simulink model "RL_voltageControl"  (R2026a)
settings: Solver=VariableStepAuto  StopTime=2000  FixedStep=1e-5
libraries: fl_lib x3, nesl_utility x3, ee_lib x2, eePwmGenerator x1
settings Model: Creator=abhinav  LastModifiedBy=abhinav
settings DataIOCC: SaveFormat=StructureWithTime

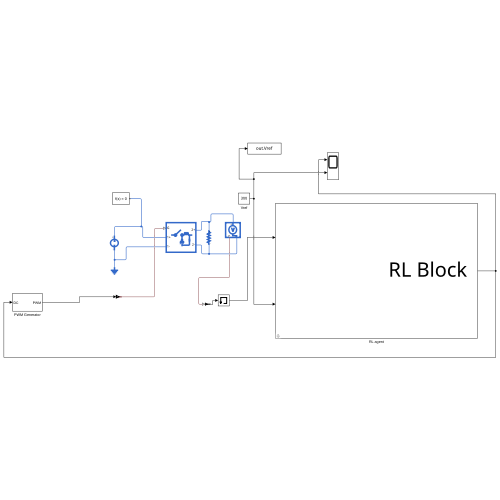
[thumbnail: Simulink's stored preview of the top-level diagram]
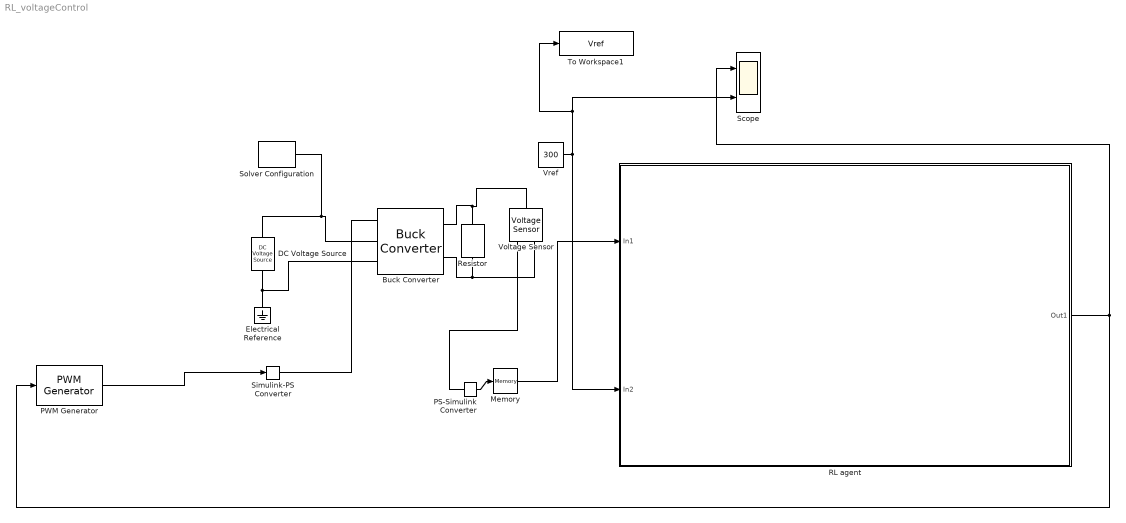
== system RL_voltageControl ==
  Buck Converter : ee_lib/Semiconductors & Converters/Converters/Buck Converter  port_option=ee.enum.controlport.ps  device_type=ee.enum.converters.switchingdevice.ideal  Vf=0.8 V  Ron=0.001 Ohm  Rds=0.001 Ohm  Goff=1e-5 1/Ohm  Vgt=1 V  Vgt_off=-1 V  Ih=1 A  Vth=6 V  K=0  diode_param=ee.enum.converters.protectiondiode.nodynamics  diode_Vf=0.8 V  diode_Ron=0.001 Ohm  diode_Goff=1e-5 1/Ohm  diode_C=50 nF  diode_iRM=-235 A  diode_iF=300 A  diode_idot=-50 A/us  diode_trr_param=ee.enum.converters.diodetrr.trr_factor  diode_trr_factor=3  diode_trr=15 us  diode_Qrr=1500 s*uA  Lf=1e-6 H  Rl=0 Ohm  Cf=1e-7 F  Rf=1e-6 Ohm  snubber_type=ee.enum.converters.snubber.exclude  Cs=1e-7 F  Rs=0.1 Ohm  iL_specify=off  iL_priority=High  iL=0 A  iL_nominal_specify=off  iL_nominal_value=1  iL_nominal_unit=A  vc_specify=off  vc_priority=High  vc=0 V  vc_nominal_specify=off  vc_nominal_value=1  vc_nominal_unit=V
  DC Voltage Source : ee_lib/Additional Components/SPICE Sources/DC Voltage Source  DC=500 V
  Electrical Reference : fl_lib/Electrical/Electrical Elements/Electrical Reference
  Memory : Memory
  PS-Simulink Converter : nesl_utility/PS-Simulink Converter  PhysicalDomain=network_engine_domain  SubClassName=ps_output  LeftPortType=input  RightPortType=output  PseudoPeriodic=off  Frequencies=[]  VectorFormat=inherit  Unit=inherit  AffineConversion=off
  PWM Generator : eePwmGenerator/PWM Generator  CarrCount=Up  Tper=0.01  Tdelay=0  Ts=1e-5
  RL agent : Subsystem  mask{Parameter1=0}
  Resistor : fl_lib/Electrical/Electrical Elements/Resistor  R=1 Ohm  i_specify=off  i_priority=None  i=0 A  i_nominal_specify=off  i_nominal_value=1  i_nominal_unit=A  v_specify=off  v_priority=None  v=0 V  v_nominal_specify=off  v_nominal_value=1  v_nominal_unit=V
  Scope : Scope  NumInputPorts=2
      settings: ActiveDisplayYMinimum=154.82767756144224  ActiveDisplayYMaximum=316.13025804872865
  Simulink-PS Converter : nesl_utility/Simulink-PS Converter  PhysicalDomain=network_engine_domain  SubClassName=ps_input  LeftPortType=input  RightPortType=output  PseudoPeriodic=off  Frequencies=[]  NoiseDistribution=none  NoiseParameters=[]  Unit=1  AffineConversion=off  FilteringAndDerivatives=provide  SimscapeFilterOrder=1  InputFilterTimeConstant=0.001  UdotUserProvided=0
  Solver Configuration : nesl_utility/Solver Configuration  PhysicalDomain=network_engine_domain  SubClassName=solver  LeftPortType=input  RightPortType=generic  Tones=[]  Harmonics=[]  SimulateNoise=off  Profile=off  UseLocalSampling=off  EnableSwitchedLinearOptims=on  FrequencyDomain=off  UseCCode=off  RelTol=0.001  AbsTol=0.001  MinStep=1e-09  ToWorkspace=off  RevertToSquareIcSolve=off  NumHomotopyIterations=100  PhasorMode=off  PhasorModeNumHarmonics=1  ConsistencySolver=NEWTON_XTOL_AFTER_FTOL  CanonicalOrdering=CANONICAL  OptimizeIntermediates=OPTIMIZED  IndexReductionMethod=DerivativeReplacement  DoDC=off  ResidualTolerance=1e-09  ConsistencyTolSource=GLOBAL  ConsistencyAbsTol=0.001  ConsistencyRelTol=0.001  ConsistencyTolFactor=0.001  UseLocalSolver=off  LocalSolverChoice=NE_BACKWARD_EULER_ADVANCER  ResolveIndetEquations=on  FunctionEvalNumThread=1  LocalSolverSampleTime=0.001  DoFixedCost=off  MaxNonlinIter=3  MaxModeIter=2  ComputeImpulses=off  ImpulseIterations=2  LinearAlgebra=auto  LinearAlgebraNumThread=0  EquationFormulation=NE_TIME_EF  DelaysMemoryBudget=1024  AutomaticFiltering=on  FilteringTimeConstant=0.001  PartitionStorageMethod=AS_NEEDED  PartitionMemoryBudget=1024  PartitionMethod=ROBUST  MultibodyUseLocalSolver=off  MultibodyLocalSolverChoice=ODE1  MultibodyLocalSolverSampleTime=0.001
  To Workspace1 : ToWorkspace  VariableName=Vref  SampleTime=-1
  Voltage Sensor : fl_lib/Electrical/Electrical Sensors/Voltage Sensor
  Vref : Constant  Value=300
  wires:
  PS-Simulink Converter/1 -> Memory/1
  PWM Generator/1 -> Simulink-PS Converter/1
  Memory/1 -> RL agent/1(In1)
  Vref/1 -> Scope/2, To Workspace1/1, RL agent/2(In2)
  RL agent/1(Out1) -> PWM Generator/1, Scope/1
  connections:
  DC Voltage Source/LConn1 -- Solver Configuration/RConn1 -- Buck Converter/LConn2
  DC Voltage Source/RConn1 -- Buck Converter/LConn3 -- Electrical Reference/LConn1
  Buck Converter/RConn1 -- Voltage Sensor/LConn1 -- Resistor/LConn1
  Buck Converter/RConn2 -- Voltage Sensor/RConn2 -- Resistor/RConn1
  Voltage Sensor/RConn1 -- PS-Simulink Converter/LConn1
  Simulink-PS Converter/RConn1 -- Buck Converter/LConn1

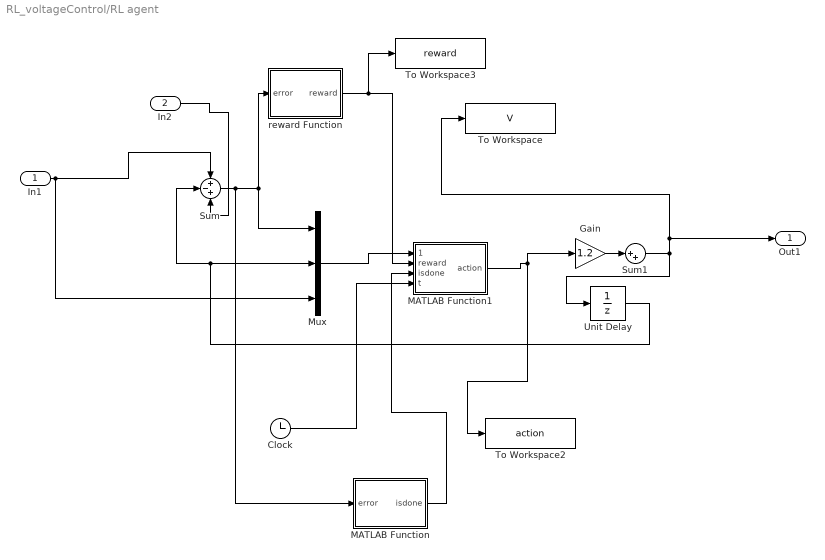
== system RL_voltageControl/RL agent ==
  In1 : Inport
  In2 : Inport  Port=2
  Clock : Clock
  Gain : Gain  Gain=1.2
  MATLAB Function : MATLAB Function  TreatAsAtomicUnit=on
  MATLAB Function1 : MATLAB Function  TreatAsAtomicUnit=on  SystemSampleTime=0.01
  Mux : Mux  Inputs=3
  Sum : Sum  Inputs=+-+
  Sum1 : Sum  Inputs=|++
  To Workspace : ToWorkspace  VariableName=V  SampleTime=-1
  To Workspace2 : ToWorkspace  VariableName=action  SampleTime=-1
  To Workspace3 : ToWorkspace  VariableName=reward  SaveFormat=Timeseries  SampleTime=-1
  Unit Delay : UnitDelay
  reward Function : MATLAB Function  TreatAsAtomicUnit=on
  Out1 : Outport
  wires:
  Clock/1 -> MATLAB Function1/4(t)
  Gain/1 -> Sum1/1
  MATLAB Function/1(isdone) -> MATLAB Function1/3(isdone)
  In1/1 -> Sum/1, Mux/3
  reward Function/1(reward) -> MATLAB Function1/2(reward), To Workspace3/1
  Mux/1 -> MATLAB Function1/1(observation)
  Unit Delay/1 -> Mux/2, Sum/2
  MATLAB Function1/1(action) -> To Workspace2/1, Gain/1
  Sum1/1 -> Out1/1, To Workspace/1, Unit Delay/1
  Sum/1 -> MATLAB Function/1(error), Mux/1, reward Function/1(error)
  In2/1 -> Sum/3

== matlab function RL_voltageControl/RL agent/MATLAB Function ==
  data: error input; isdone output
function isdone = fcn(error)
isdone = abs(error) > 350;
end
%#codegen

== matlab function RL_voltageControl/RL agent/reward Function ==
  data: error input; reward output

%#codegen
function reward = fcn(error)
    reward = -error^2;
end

== matlab function RL_voltageControl/RL agent/MATLAB Function1 ==
  settings: updateMethod=DISCRETE
  data: observation input; action output; reward input; isdone input; t input
function action = fcn(observation, reward, isdone, t)
persistent W b bestW bestb bestReward totalReward episodeStartTime

if isempty(W)
    W = 0.01 * randn(1,3);
    b = 150;
    bestW = W; bestb = b;
    bestReward = -Inf;
    totalReward = 0;
    episodeStartTime = 0;
end

obsNorm = observation / 300;
action = W * obsNorm + b;
action = min(max(action, 0), 350);

totalReward = totalReward + reward;

episodeLength = 10;   % seconds per "episode"
episodeEnd = (t - episodeStartTime) >= episodeLength;

if episodeEnd
    if totalReward > bestReward
        bestReward = totalReward;
        bestW = W;
        bestb = b;
    else
        W = bestW;
        b = bestb;
    end

    W = bestW + 0.5*randn(size(bestW));
    b = bestb + 5*randn;

    totalReward = 0;
    episodeStartTime = t;
end
end
